simulink model "tb_per_tebvfh_top"  (R2026b)
undefined symbols (not defined in the file or in its folder): Ts
settings Model: Creator=aomar  LastModifiedBy=aomar

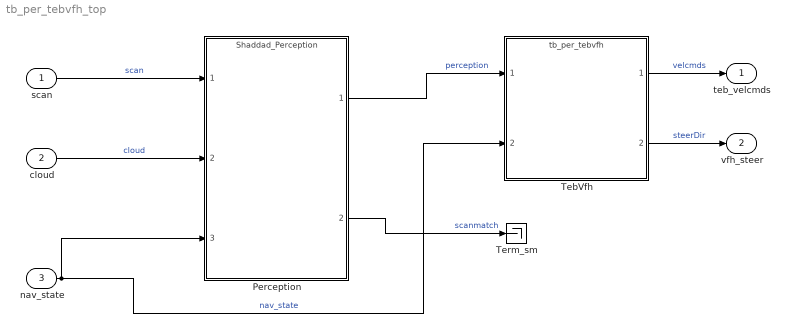
== system tb_per_tebvfh_top ==
  scan : Inport  OutDataTypeStr=Bus: Bus_LidarScanRaw  SampleTime=Ts.lidar  Interpolate=off
  cloud : Inport  Port=2  OutDataTypeStr=Bus: Bus_LidarCloudRaw  SampleTime=Ts.lidar  Interpolate=off
  nav_state : Inport  Port=3  OutDataTypeStr=Bus: Bus_NavState  SampleTime=Ts.nav  Interpolate=off
  Perception : ModelReference  ModelNameDialog=Shaddad_Perception  SimulationMode=Normal  ModelReferenceVersion=1.1
  TebVfh : ModelReference  ModelNameDialog=tb_per_tebvfh  ModelReferenceVersion=1.1
  Term_sm : Terminator
  teb_velcmds : Outport
  vfh_steer : Outport  Port=2
  wires:
  scan/1 -> Perception/1  "scan"
  cloud/1 -> Perception/2  "cloud"
  nav_state/1 -> TebVfh/2, Perception/3  "nav_state"
  Perception/1 -> TebVfh/1  "perception"
  Perception/2 -> Term_sm/1  "scanmatch"
  TebVfh/1 -> teb_velcmds/1  "velcmds"
  TebVfh/2 -> vfh_steer/1  "steerDir"
